simulink model "fuzzy_stepmotor_casa"  (Simulink 7.0)
settings: Solver=FixedStepDiscrete  StartTime=0.0  StopTime=10.0  FixedStep=0.001  RelTol=1e-3
undefined symbols (not defined in the file or in its folder): DiscIntNeverNeededParam
libraries: simulink x6, dsPICdrivers x4, dspswit3 x1, fuzblock x1
settings Model: Creator=ALAN  LastModifiedBy=ALAN-PC
settings OptimizationCC: OptimizeModelRefInitCode=on  LifeSpan=1
settings HardwareCC: ProdBitPerInt=16  ProdEndianess=LittleEndian  ProdWordSize=16  ProdHWDeviceType=16-bit Generic  TargetHWDeviceType=32-bit Generic
settings RTWCC: SystemTargetFile=dspic.tlc  TemplateMakefile=dspic_pic30_gcc.tmf  PostCodeGenCommand=dsPIC_Compile()  Description=Embedded Target for Microchip dsPIC (real-time)  ProcessScript=dspic_make_rtw_hook
settings CodeAppCC: IgnoreCustomStorageClasses=off
settings STFCustomTargetCC: GenFloatMathFcnCalls=ANSI_C  ModelReferenceCompliant=off  IncludeMdlTerminateFcn=off  CombineOutputUpdateFcns=on  SuppressErrorStatus=on  ERTCustomFileBanners=on  SupportContinuousTime=off  SupportNonInlinedSFcns=off  SystemTargetFile=dspic.tlc
settings ERTTargetCC: GenFloatMathFcnCalls=ANSI_C  ModelReferenceCompliant=off  CompOptLevelCompliant=off  IncludeMdlTerminateFcn=off  SuppressErrorStatus=on  ModelStepFunctionPrototypeControlCompliant=off  ExtModeMexFile=noextcomm  InlinedParameterPlacement=NonHierarchical  ERTSrcFileBannerTemplate=dsPIC_code_template.cgt  ERTHdrFileBannerTemplate=dsPIC_code_template.cgt  ERTDataSrcFileTemplate=dsPIC_code_template.cgt  ERTDataHdrFileTemplate=dsPIC_code_template.cgt  ERTCustomFileTemplate=dsPIC_main.tlc
settings CustomProperty: DataType=string  Value=E:\ARQUIV~1\MATLAB\R2007b\bin\win32\gmake

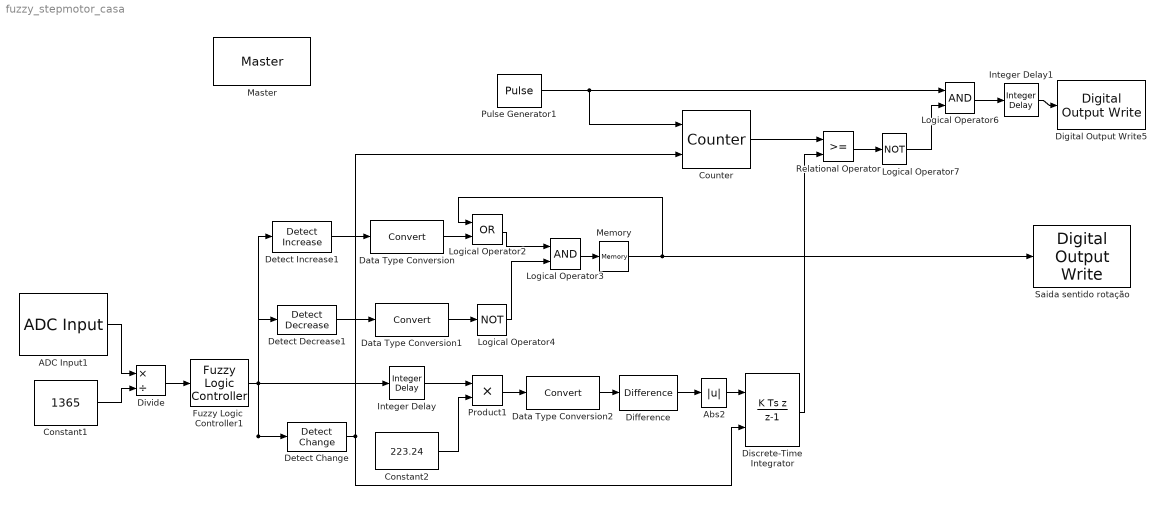
== system fuzzy_stepmotor_casa ==
  ADC Input1 : dsPICdrivers/Peripheral I//O/ADC Input  Tag=dsPIC_ADC  Priority=5  ADC_TYPE=12 bits  ADC_MODE=Continuous sampling & get last channel value  NbrSampleStep=1  VoltRefpopup="AVdd  -  AVss"  OutFormatBitspopup=0000 dddd dddd dddd : Integer  InterruptPriority=6  ANCHANNELS=[6]  MaxName=ANmax = 4095  Rin=10000  ADCS=6  SAMC=1  Temperature=25  DMAChannel=0  SampleTime=-1  Status="OK  |  Tsmp=7.000e-007 |  T/Channel=1.050e-005 |  Tall=1.050e-005"  SSRC=auto convert
  Abs2 : Abs  OutDataType=sfix(16)  OutScaling=2^0  RndMeth=Nearest
  Constant1 : Constant  Value=1365  OutDataType=sfix(16)  OutScaling=2^0  SampleTime=-1
  Constant2 : Constant  Value=223.24  OutDataType=sfix(16)  OutScaling=2^0  SampleTime=0.001
  Counter : dspswit3/Counter  Direction=Up  CountEvent=Rising edge  CounterSize=User defined  MaxCount=9999999999999999999999  InitialCount=0  Output=Count  HitValue=32  ResetInput=on  SamplesPerFrame=1  Ts=1  CntDtype=double  HitDtype=Logical
  Data Type Conversion : DataTypeConversion  OutDataTypeMode=boolean  OutDataType=sfix(16)  OutScaling=2^0  SampleTime=0.001
  Data Type Conversion1 : DataTypeConversion  OutDataTypeMode=boolean  OutDataType=sfix(16)  OutScaling=2^0
  Data Type Conversion2 : DataTypeConversion  OutDataTypeMode=int16  OutDataType=sfix(16)  OutScaling=2^0  RndMeth=Nearest
  Detect Change : simulink/Logic and Bit Operations/Detect Change  SystemSampleTime=-1  vinit=0
  Detect Decrease1 : simulink/Logic and Bit Operations/Detect Decrease  SystemSampleTime=-1  vinit=0.0
  Detect Increase1 : simulink/Logic and Bit Operations/Detect Increase  SystemSampleTime=-1  vinit=0.0
  Difference : simulink/Discrete/Difference  SystemSampleTime=-1  ICPrevInput=0.0  OutMin=[]  OutMax=[]  OutDataType=sfix(16)  OutScaling=2^-10  DoSatur=off
  Digital Output Write5 : dsPICdrivers/Digital I//O/Digital Output Write  Tag=dsPIC_Digital_Output  Priority=5  PORT=B  Pin=[0]  Simultaneous=on  OrderingInOutPopup=None
  Discrete-Time Integrator : DiscreteIntegrator  IntegratorMethod=Integration: Backward Euler  gainval=1000  ExternalReset=rising  SampleTime=0.001  OutDataType=sfix(16)  OutScaling=2^0  RndMeth=Nearest  ICPrevOutput=DiscIntNeverNeededParam  ICPrevScaledInput=DiscIntNeverNeededParam
  Divide : Product  Inputs=*/  OutDataTypeMode=double  OutDataType=sfix(16)  OutScaling=2^-10
  Fuzzy Logic  Controller1 : fuzblock/Fuzzy Logic  Controller  SystemSampleTime=-1  fis=lente_act3
  Integer Delay : simulink/Discrete/Integer Delay  vinit=0.0  samptime=-1  NumDelays=1
  Integer Delay1 : simulink/Discrete/Integer Delay  vinit=0.0  samptime=-1  NumDelays=1
  Logical Operator2 : Logic  Operator=OR  OutDataTypeMode=boolean
  Logical Operator3 : Logic  AllPortsSameDT=off  OutDataTypeMode=boolean
  Logical Operator4 : Logic  Operator=NOT  AllPortsSameDT=off  OutDataTypeMode=boolean
  Logical Operator6 : Logic  AllPortsSameDT=off  OutDataTypeMode=boolean
  Logical Operator7 : Logic  Operator=NOT  AllPortsSameDT=off  OutDataTypeMode=boolean
  Master : dsPICdrivers/Master  Tag=dsPIC_MASTER  Priority=1  TimeStepType=Timer1  picType=30f3012  fcy=5e6  Quartz_33f=5e6  PLLActive_33f=off  fcyDesired_33f=0  tmr1="[1  4999  0]"  tmr1Info="Time Step : 0.001  ;   Error : 0%  PR1=4999"  tmr2345="[0  0]"  tmr2345cfg=[-1 -1]  IOautoConf=on  typePort="[ 0   0   0   0   0   0   0   0   0   0   0   0   0   0   0   0  10   0  10   0   0   0   8   0   0   0   0   0   0   0   0   0   0   0   0   0   0   0   0   0   0   0   0   0   0   0   0   0   0   0   0   0   0   0   0   0   0   0   0   0   0   0   0   0   0   0   0   0   0   0   0   0   0   0   0   0   0   0   0   0   0   0   0   0   0   0   0   0   0   0   0   0   0   0   0   0   0   0   0   0   0   0   0   0   0   0   0   0   0   0   0   0 ]"  TRIS="[ 65535  65530  65535  65535  65535  65535  65535 ]"  ADPCFG=5  MasterBusyPort=None  MasterOverloadPort=None  FOSC=HS  ClockSwitchMonitor=Both disabled  TempProtection_33f=TEMP_ON  FPBOR=PBOR_OFF  PWRT=PWRT_OFF  MCLR=MCLR_DIS  PowerSave=off  OverrideFcy=off  NewFcy=1e6  PR2345="[65535  65535]"
  Memory : Memory
  Product1 : Product  OutDataType=sfix(16)  OutScaling=2^0  RndMeth=Zero
  Pulse Generator1 : DiscretePulseGenerator  PulseType=Time based  Period=0.01  PulseWidth=50
  Relational Operator : RelationalOperator  LogicOutDataTypeMode=boolean
  Saida sentido rotação : dsPICdrivers/Digital I//O/Digital Output Write  Tag=dsPIC_Digital_Output  Priority=5  PORT=B  Pin=[2]  Simultaneous=on  OrderingInOutPopup=None
  wires:
  Constant1/1 -> Divide/2
  ADC Input1/1 -> Divide/1
  Fuzzy Logic  Controller1/1 -> Detect Change/1, Detect Decrease1/1, Detect Increase1/1, Integer Delay/1
  Detect Increase1/1 -> Data Type Conversion/1
  Detect Decrease1/1 -> Data Type Conversion1/1
  Detect Change/1 -> Counter/2, Discrete-Time Integrator/2
  Logical Operator4/1 -> Logical Operator3/2
  Data Type Conversion1/1 -> Logical Operator4/1
  Logical Operator3/1 -> Memory/1
  Logical Operator2/1 -> Logical Operator3/1
  Memory/1 -> Saida sentido rotação/1, Logical Operator2/1
  Pulse Generator1/1 -> Logical Operator6/1, Counter/1
  Constant2/1 -> Product1/2
  Product1/1 -> Data Type Conversion2/1
  Data Type Conversion2/1 -> Difference/1
  Counter/1 -> Relational Operator/1
  Relational Operator/1 -> Logical Operator7/1
  Difference/1 -> Abs2/1
  Discrete-Time Integrator/1 -> Relational Operator/2
  Integer Delay/1 -> Product1/1
  Logical Operator7/1 -> Logical Operator6/2
  Abs2/1 -> Discrete-Time Integrator/1
  Logical Operator6/1 -> Integer Delay1/1
  Integer Delay1/1 -> Digital Output Write5/1
  Divide/1 -> Fuzzy Logic  Controller1/1
  Data Type Conversion/1 -> Logical Operator2/2
